simulink model "FMS"  (R2018b)
settings: configuration reference "fms_config" (kept outside this file)
values from neighbouring files (symbols this model uses):
  FMS_EXPORT = Simulink.Parameter(FMS_EXPORT_VALUE)    [fms_model_init.m]
  FMS_PARAM = Simulink.Parameter(FMS_PARAM_VALUE)    [fms_model_init.m]
undefined symbols (not defined in the file or in its folder): actuator_cmd, cmd_mask, ControlMode, ctrl_mode, DiscIntNeverNeededParam, FMS_Cmd, FMS_CONST, home, mode, PilotMode, r_cmd, reset, state, status, timestamp, u_cmd, VehicleState, VehicleStatus, wp_consume, wp_current
libraries: simulink x45, FMT_Model_Lib x35, hdlsllib x2
(part 3 of 3)

== system FMS/FMS Commander/Commander/Arm/Assist/Position/Position Command/Controller/Hold Control/Lateral_Acceleration/L1_Lateral_Acceleration/Included Angle ==
  vec1 : Inport
  vec2 : Inport  Port=2
  2D Cross Product : FMT_Model_Lib/Math/2D Cross Product
      settings: SourceProductName=FMT Toolbox
  Acos : Trigonometry  Operator=acos
  Constant4 : Constant  OutDataTypeStr=single
  Demux : Demux  Outputs=2
  Demux1 : Demux  Outputs=2
  Dot Product : DotProduct  InputSameDT=on  OutDataTypeStr=Inherit: Inherit via internal rule
  Multiply : Product
  Mux : Mux  Inputs=2
  Mux1 : Mux  Inputs=2
  Sign1 : Signum
  Switch2 : Switch  Criteria=u2 ~= 0
  Vector Normalize : FMT_Model_Lib/Math/Vector Normalize
      settings: SourceProductName=FMT Toolbox
  Vector Normalize1 : FMT_Model_Lib/Math/Vector Normalize
      settings: SourceProductName=FMT Toolbox
  angle_rad : Outport
  wires:
  Switch2/1 -> Multiply/2
  Acos/1 -> Multiply/1
  Mux/1 -> Vector Normalize1/1
  vec2/1 -> Demux/1
  Constant4/1 -> Switch2/3
  Demux/1 -> Mux/2
  vec1/1 -> Demux1/1
  Multiply/1 -> angle_rad/1
  2D Cross Product/1 -> Sign1/1
  Vector Normalize/1 -> 2D Cross Product/2, Dot Product/1
  Demux/2 -> Mux/1
  Vector Normalize1/1 -> 2D Cross Product/1, Dot Product/2
  Sign1/1 -> Switch2/2, Switch2/1
  Demux1/2 -> Mux1/1
  Mux1/1 -> Vector Normalize/1
  Demux1/1 -> Mux1/2
  Dot Product/1 -> Acos/1

== matlab function FMS/FMS Commander/Commander/Arm/SubMode/Return/Velocity Commander/L1 Reference WP/NearbyRefWP ==
  data: P output; P2 input; d output; P3 input; L1 input
% Find the reference waypoint when vehicle (P3) is close to target (P2)
%
% If the vehicle is close to target (distance(P2,P3) < L1), select P2 as
% reference waypoint and return the distance, otherwise return -1.
function [P,d] = NearbyRefWP(P2, P3, L1)

P3P2 = P2 - P3;
dis = sqrt(sum(P3P2.^2));

if dis <= L1
    d = dis;
    % select P2 as reference WP
    P = P2;
else
    d = single(-1);
    % unset WP
    P = single([0; 0]);
end

== matlab function FMS/FMS Commander/Commander/Arm/SubMode/Return/Velocity Commander/L1 Reference WP/OutRegionRegWP ==
  data: P1 input; P output; P2 input; P3 input
% Find the reference waypoint when vehicle is out of L1 region near P1P2.
%
% There are three region defined:
%   Region 1: The project point of P3 is lied on left side of P1P2
%   Region 2: The project point of P3 is lied on right side of P1P2
%   Region 3: The project point of P3 is lied on the segment line 
%
%   For the case of region 3, we select the project point as the reference
%   wayspoint. For the case of region 1, we choose P1 as reference waypoint
%   and similarly for the case of region 2, we choose P3 as reference
%   waypoint.
function P = OutRegionRefWP(P1, P2, P3)
% segment line P1P2
P1P2 = P2 - P1;
% segment line P1P3
P1P3 = P3 - P1;

% Define C as the P3 project point on line P1P2.
% Hence, P1C = dot(P1P3, P1P2)/|P1P2| * (P1P2/|P1P2|) = u * P1P2
% where u = dot(P1P3, P1P2) / |P1P2|^2.
u = dot(P1P3, P1P2) / sum(P1P2.^2);

if u <= 0
    % region 1
    P = P1;
elseif u >= 1
    % region 2
    P = P2;
else
    % region 3. C = P1C + P1
    P = u * P1P2 + P1;
end

== stateflow chart FMS/SafeMode ==
  state Other
  state Offboard
  state Mission
  state Position
  state Stabilize
  state Manual
  (junction 21) -> Other
  Other -> (junction 68) : {target_mode = mode;}
  (junction 75) -> (junction 21) [order 2]
  (junction 68) -> (junction 84)
  Offboard -> (junction 78)
  (junction 78) -> (junction 84) [order 1] : [bitget(flag, 4)&&bitget(flag, 5)]
      | {target_mode = PilotMode.Offboard;}
  (junction 75) -> Offboard [order 1] : [mode == PilotMode.Offboard]
  (junction 78) -> (junction 88) [order 2]
  (junction 84) -> (junction 48)
  (junction 1) -> (junction 75) [order 2]
  (junction 1) -> Mission [order 1] : [mode == PilotMode.Mission]
  Mission -> (junction 16)
  (junction 16) -> (junction 48) [order 1] : [bitget(flag, 4)&&bitget(flag, 6)]
      | {target_mode = PilotMode.Mission;}
  (junction 16) -> (junction 88) [order 2]
  (junction 47) -> (junction 1) [order 2]
  (junction 48) -> (junction 51)
  (junction 47) -> Position [order 1] : [mode == PilotMode.Position]
  Position -> (junction 49)
  (junction 49) -> (junction 51) [order 1] : [bitget(flag, 4)&&bitget(flag, 7)]
      | {target_mode = PilotMode.Position;}
  (junction 49) -> (junction 88) [order 2]
  (junction 24) -> (junction 47) [order 2]
  (junction 51) -> (junction 39)
  (junction 88) -> Stabilize
  (junction 24) -> Stabilize [order 1] : [mode == PilotMode.Stabilize]
  Stabilize -> (junction 44)
  (junction 44) -> (junction 39) [order 1] : [bitget(flag, 4)]{target_mode = PilotMode.Stabilize;}
  (junction 44) -> Manual [order 2]
  (junction 10) -> (junction 24) [order 1]
  (junction 39) -> (junction 15)
  (default) -> (junction 10)
  (junction 10) -> Manual [order 2] : [mode == PilotMode.Manual]
  Manual -> (junction 15) : {target_mode = PilotMode.Manual;}
  (junction 41) -> (junction 10)
  (junction 15) -> (junction 40)
  (junction 40) -> (junction 41)
  data: target_mode output; mode input Enum: PilotMode; flag input uint32

== matlab function FMS/FMS Commander/Commander/Arm/SubMode/Return/Velocity Commander/L1 Reference WP/SearchL1RefWP ==
  data: P1 input; P output; P2 input; P3 input; L1 input; u output
% Find reference waypoint (L1RefWP) on the line segment P1P2 which has 
% L1 distance from vehicle position (P3).
%
% The idea is to calculate the intersection point of a circle with L1 radius
% with the line segment P1P2.
%
% Define P = P1 + u * (P2 - P1), where P is the intersection point.
% Goal is calculating the u, where the valid u is between [0, 1].
%
% Input:
%   P1: start point of segment line
%   P2: start point of segment line
%   P3: circle center point, also is known as the vehicle position
%   L1: the L1 distance
% Output:
%   P: L1 reference waypoint
%   u: scale factor (valid between 0 and 1), -1 means no intersection.
function [P, u] = SearchL1RefWP(P1, P2, P3, L1)

% P1 = (x1, y1), P2 = (x2, y2), P3 = (x3, y3)
x1 = P1(1);
y1 = P1(2);
x2 = P2(1);
y2 = P2(2);
x3 = P3(1);
y3 = P3(2);

% The P is on circle and line segment, which yields:
A = (x2 - x1)^2 + (y2 - y1)^2;
B = 2 * ((x2 - x1)*(x1 - x3) + (y2 - y1)*(y1 - y3));
C = x3^2 + y3^2 + x1^2 + y1^2 - 2*(x3*x1 + y3*y1) - L1^2;
% Check root existence confition if B^2 - 4*A*C >= 0
D = B^2 - 4*A*C;
u = single(-1);
P = single([0 0]);

if D > 0
    % D>0 means we have 2 difference roots, % root is valid only if u is in range of [0, 1]
    u1 = (-B + sqrt(D)) / (2*A);
    u2 = (-B - sqrt(D)) / (2*A);
    
    if (u1>=0 && u1<=1) && (u2>=0 && u2<=1)
        % have 2 valid roots, select the one which is closer to P2 (target point)
        if u1 > u2
            u = u1; 
        else
            u = u2;
        end
    elseif (u1>=0 && u1<=1)
        % only 1 root valid, select it
        u = u1;
    elseif (u2>=0 && u2<=1)
        % only 1 root valid, select it
        u = u2;
    else
        % no valid root, which means no intersection point founded.
        return;
    end
elseif D == 0
    % D=0 means only 1 single root
    u1 = -B / (2*A);
    if (u1>=0 && u1<=1)
        % valid root, select it
        u = u1;
    else
        % no valid root, which means no intersection point founded.
        return;
    end
else
    % no valid root, which means no intersection point founded.
    return;
end

% calculate the L1 reference waypoint (P) coordinate
P(1) = x1 + u*(x2 - x1);
P(2) = y1 + u*(y2 - y1);

== matlab function FMS/FMS Commander/Commander/Arm/Auto/Mission/Mission_SubSystem/Velocity Commander/L1 Reference WP/NearbyRefWP ==
  data: P output; P2 input; d output; P3 input; L1 input
% Find the reference waypoint when vehicle (P3) is close to target (P2)
%
% If the vehicle is close to target (distance(P2,P3) < L1), select P2 as
% reference waypoint and return the distance, otherwise return -1.
function [P,d] = NearbyRefWP(P2, P3, L1)

P3P2 = P2 - P3;
dis = sqrt(sum(P3P2.^2));

if dis <= L1
    d = dis;
    % select P2 as reference WP
    P = P2;
else
    d = single(-1);
    % unset WP
    P = single([0; 0]);
end

== matlab function FMS/FMS Commander/Commander/Arm/Auto/Mission/Mission_SubSystem/Velocity Commander/L1 Reference WP/OutRegionRegWP ==
  data: P1 input; P output; P2 input; P3 input
% Find the reference waypoint when vehicle is out of L1 region near P1P2.
%
% There are three region defined:
%   Region 1: The project point of P3 is lied on left side of P1P2
%   Region 2: The project point of P3 is lied on right side of P1P2
%   Region 3: The project point of P3 is lied on the segment line 
%
%   For the case of region 3, we select the project point as the reference
%   wayspoint. For the case of region 1, we choose P1 as reference waypoint
%   and similarly for the case of region 2, we choose P3 as reference
%   waypoint.
function P = OutRegionRefWP(P1, P2, P3)
% segment line P1P2
P1P2 = P2 - P1;
% segment line P1P3
P1P3 = P3 - P1;

% Define C as the P3 project point on line P1P2.
% Hence, P1C = dot(P1P3, P1P2)/|P1P2| * (P1P2/|P1P2|) = u * P1P2
% where u = dot(P1P3, P1P2) / |P1P2|^2.
u = dot(P1P3, P1P2) / sum(P1P2.^2);

if u <= 0
    % region 1
    P = P1;
elseif u >= 1
    % region 2
    P = P2;
else
    % region 3. C = P1C + P1
    P = u * P1P2 + P1;
end

== matlab function FMS/FMS Commander/Commander/Arm/Auto/Mission/Mission_SubSystem/Velocity Commander/L1 Reference WP/SearchL1RefWP ==
  data: P1 input; P output; P2 input; P3 input; L1 input; u output
% Find reference waypoint (L1RefWP) on the line segment P1P2 which has 
% L1 distance from vehicle position (P3).
%
% The idea is to calculate the intersection point of a circle with L1 radius
% with the line segment P1P2.
%
% Define P = P1 + u * (P2 - P1), where P is the intersection point.
% Goal is calculating the u, where the valid u is between [0, 1].
%
% Input:
%   P1: start point of segment line
%   P2: start point of segment line
%   P3: circle center point, also is known as the vehicle position
%   L1: the L1 distance
% Output:
%   P: L1 reference waypoint
%   u: scale factor (valid between 0 and 1), -1 means no intersection.
function [P, u] = SearchL1RefWP(P1, P2, P3, L1)

% P1 = (x1, y1), P2 = (x2, y2), P3 = (x3, y3)
x1 = P1(1);
y1 = P1(2);
x2 = P2(1);
y2 = P2(2);
x3 = P3(1);
y3 = P3(2);

% The P is on circle and line segment, which yields:
A = (x2 - x1)^2 + (y2 - y1)^2;
B = 2 * ((x2 - x1)*(x1 - x3) + (y2 - y1)*(y1 - y3));
C = x3^2 + y3^2 + x1^2 + y1^2 - 2*(x3*x1 + y3*y1) - L1^2;
% Check root existence confition if B^2 - 4*A*C >= 0
D = B^2 - 4*A*C;
u = single(-1);
P = single([0 0]);

if D > 0
    % D>0 means we have 2 difference roots, % root is valid only if u is in range of [0, 1]
    u1 = (-B + sqrt(D)) / (2*A);
    u2 = (-B - sqrt(D)) / (2*A);
    
    if (u1>=0 && u1<=1) && (u2>=0 && u2<=1)
        % have 2 valid roots, select the one which is closer to P2 (target point)
        if u1 > u2
            u = u1; 
        else
            u = u2;
        end
    elseif (u1>=0 && u1<=1)
        % only 1 root valid, select it
        u = u1;
    elseif (u2>=0 && u2<=1)
        % only 1 root valid, select it
        u = u2;
    else
        % no valid root, which means no intersection point founded.
        return;
    end
elseif D == 0
    % D=0 means only 1 single root
    u1 = -B / (2*A);
    if (u1>=0 && u1<=1)
        % valid root, select it
        u = u1;
    else
        % no valid root, which means no intersection point founded.
        return;
    end
else
    % no valid root, which means no intersection point founded.
    return;
end

% calculate the L1 reference waypoint (P) coordinate
P(1) = x1 + u*(x2 - x1);
P(2) = y1 + u*(y2 - y1);

== stateflow chart FMS/FMS Commander/Commander/Arm/Assist/Stabilize/Heading Command/Detect Movement/Motion State ==
  state Hold
    entry:
    state=MotionState.Hold;
  state Move
    entry:
    state=MotionState.Move;
  state Brake
    entry:
    state=MotionState.Brake;
  (default) -> Move
  Hold -> Move : [motion_req==1 ]
  Move -> Brake : [motion_req==0]
  Brake -> Move [order 1] : [motion_req==1]
  Brake -> Hold [order 2] : after(1.5, sec)
  data: state output Enum: MotionState; motion_req input

== stateflow chart FMS/FMS State Machine ==
  state Command_Listener [parallel]
    settings: executionOrder=1
    state Send
      entry:
      % Send command
      M.data=save_cmd;
      send(M);
    state Listen
    state Check
      entry:
      valid_cmd = CheckCmdValid(save_cmd, mode, INS_Out.flag);
    (default) -> Listen
    Send -> Listen
    Listen -> Check : [hasChanged(cmd) && ...
        | cmd ~= FMS_Cmd.None]{save_cmd = cmd;}
    Check -> Listen [order 2]
    Check -> Send [order 1] : [valid_cmd == true]
  state Vehicle [parallel]
    du:
    % if mission data updated, reset waypoint index
    if hasChanged(mission_timestamp)
    wp_consume = 0;
    wp_index = 1;
    end
    settings: executionOrder=4
    state moved = StickMoved(stick_val,pilot_cmd) [function]
    state Arm
      en:
      status = VehicleStatus.Arm;
      state SubMode
        en:
        stick_val = [Pilot_Cmd.stick_yaw; Pilot_Cmd.stick_throttle; Pilot_Cmd.stick_roll; Pilot_Cmd.stick_pitch];
        state Hold
          en:
          state = VehicleState.Hold;
        state Return
          en:
          state = VehicleState.Return;
        SubMode -> Hold [order 1] : M[M.data==FMS_Cmd.Pause]
      state Auto
        state Offboard
          state Loiter
            en:
            state = VehicleState.Hold;
          state Run
            en:
            state = VehicleState.Offboard;
          (default) -> (junction 950)
          (junction 950) -> Vehicle.Arm.Auto.Offboard.Loiter [order 2]
          (junction 950) -> Run [order 1] : [auto_cmd_valid == 1]
          Run -> Vehicle.Arm.Auto.Offboard.Loiter : [auto_cmd_valid == 0]
          Vehicle.Arm.Auto.Offboard.Loiter -> Run : [auto_cmd_valid == 1]
        state Mission
          en:
          % Reference location of latitude and longitude, specified as an m-by-2 array, in degrees
          llo = [INS_Out.lat_0, INS_Out.lon_0] * (180/pi);
          Cmd_In.cur_waypoint =[INS_Out.x_R; INS_Out.y_R; INS_Out.h_R];
          state pos = LLA2FLAT(lla,llo,href,psio) [function]
          state Loiter
            en:
            state = VehicleState.Hold;
          state NextWP
            en:
            if wp_index <= Mission_Data.valid_items
            nav_cmd = Mission_Data.command(wp_index);
            else
            nav_cmd = uint16(NAV_Cmd.None);
            % updated consumed waypoints
            wp_consume = wp_index - 1;
            end
          state Waypoint
            en:
            % Geodetic coordinates (latitude, longitude, and altitude), specified as an m-by-3 array in [degrees degrees meters]
            % Altitude add home(3) here because the altitude when takeoff could be non-zero
            lla = [double(Mission_Data.x(wp_index))*1e-7, double(Mission_Data.y(wp_index))*1e-7, double(-(Mission_Data.z(wp_index) + home(3)))];
            % target waypoint
            Cmd_In.sp_waypoint = LLA2FLAT(lla, llo, 0, 0);
            state = VehicleState.Mission;
          state Return
            en:
            Cmd_In.sp_waypoint = [home(1); home(2); INS_Out.h_R];
            state = VehicleState.Return;
          Mission -> NextWP : [hasChanged(mission_timestamp)]
          (junction 908) -> (junction 910) : {wp_index = wp_index + 1;}
          (junction 910) -> NextWP
          (junction 873) -> (junction 908)
          (default) -> NextWP
          (junction 917) -> Vehicle.Arm.Auto.Mission.Loiter
          (junction 879) -> (junction 873)
          NextWP -> (junction 917) [order 3]
          NextWP -> Waypoint [order 1] : [nav_cmd == NAV_Cmd.Waypoint]
          Waypoint -> (junction 879) : [norm([INS_Out.x_R;INS_Out.y_R]-Cmd_In.sp_waypoint(1:2)) <= accept_radius]
              | {Cmd_In.cur_waypoint = Cmd_In.sp_waypoint;}
          (junction 915) -> (junction 879)
          NextWP -> Vehicle.Arm.Auto.Mission.Return [order 2] : [nav_cmd == NAV_Cmd.Return]
          Vehicle.Arm.Auto.Mission.Return -> (junction 915) : [norm([INS_Out.x_R; INS_Out.y_R]-Cmd_In.sp_waypoint(1:2)) < 0.5]
        state InvalidAutoMode
        (default) -> (junction 43)
        (junction 43) -> Offboard [order 1] : [mode == PilotMode.Offboard]
        (junction 43) -> (junction 134) [order 2]
        (junction 134) -> Mission [order 1] : [mode == PilotMode.Mission]
        (junction 134) -> InvalidAutoMode [order 2]
        InvalidAutoMode -> (junction 370)
      state Assist
        state InvalidAssistMode
        state Stabilize
          en:
          state = VehicleState.Stabilize;
        state Position
          en:
          state = VehicleState.Position;
        (default) -> (junction 190)
        (junction 190) -> (junction 196) [order 2]
        (junction 196) -> InvalidAssistMode [order 2]
        (junction 190) -> Stabilize [order 1] : [mode == PilotMode.Stabilize]
        (junction 196) -> Position [order 1] : [mode == PilotMode.Position]
      state Manual
        state InValidManualMode
        state Manual
          en:
          state = VehicleState.Manual;
        (default) -> (junction 410)
        (junction 410) -> InValidManualMode [order 2]
        (junction 410) -> Vehicle.Arm.Manual.Manual [order 1] : [mode == PilotMode.Manual]
      state InvalidArmMode
      Vehicle.Arm -> Vehicle.Arm.SubMode.Return [order 2] : M[M.data==FMS_Cmd.Return]
          | {Cmd_In.sp_waypoint = [home(1); home(2); single(0)]}
      Hold -> Vehicle.Arm : M[M.data==FMS_Cmd.Continue ...
          | && mode ~= PilotMode.None]
      Auto -> Hold : M[M.data==FMS_Cmd.Pause]
      SubMode -> (junction 117) [order 1] : [StickMoved(stick_val, Pilot_Cmd) && ...
          | mode ~= PilotMode.None]
      Vehicle.Arm -> (junction 117) [order 1] : [hasChanged(mode) && ...
          | mode ~= PilotMode.None]
      (junction 117) -> Auto [order 1] : [getArmMode(mode) == 3]
      (default) -> (junction 117)
      (junction 117) -> (junction 140) [order 2]
      (junction 140) -> Assist [order 1] : [getArmMode(mode)  == 2]
      (junction 140) -> (junction 240) [order 2]
      (junction 240) -> Vehicle.Arm.Manual [order 1] : [getArmMode(mode)  == 1]
      (junction 240) -> InvalidArmMode [order 2]
    state Standby
      en:
      % check if mission takeoff is valid
      if mode==PilotMode.Mission
      if wp_index <= Mission_Data.valid_items > 0
      % set mission takeoff flag, so enter mission mode after 2s
      prep_mission = 1;
      else
      send(DisarmEvent);
      end
      end
      % set current position as home
      home = [INS_Out.x_R; INS_Out.y_R; INS_Out.h_R; INS_Out.psi];
      % enter standby state
      state = VehicleState.Standby;
      status = VehicleStatus.Standby;
      ex:
      % on exit, unset flag
      prep_mission = 0;
    state Disarm
      en:
      state = VehicleState.Disarm;
      status = VehicleStatus.Disarm;
    InValidManualMode -> Vehicle
    Vehicle.Arm.SubMode.Return -> (junction 330) : [norm([INS_Out.x_R,INS_Out.y_R]-[home(1),home(2)]) ...
        | <= accept_radius]
    (junction 330) -> Vehicle.Disarm
    (junction 969) -> Hold
    (junction 968) -> (junction 969) : [pilot_cmd_lost]
    InvalidAssistMode -> Vehicle
    (junction 370) -> Vehicle
    (default) -> Vehicle.Disarm
    Assist -> (junction 968)
    Standby -> Vehicle.Disarm [order 2] : after(10, sec) || DisarmEvent
    Standby -> Vehicle.Arm [order 1] : [ManualArmEvent(Pilot_Cmd) == 1 &&...
        | mode ~= PilotMode.None]
    Vehicle.Disarm -> Standby : M[M.data==FMS_Cmd.PreArm]
    Standby -> Vehicle.Arm [order 4] : [mode == PilotMode.Offboard && ...
        | auto_cmd_valid]
    Vehicle -> Vehicle.Disarm : M[M.data==FMS_Cmd.Disarm]
    Standby -> (junction 903) [order 3] : [duration(prep_mission == 1) >= 2]
    (junction 903) -> Vehicle.Arm
    InvalidArmMode -> Vehicle
  state Combo_Stick [parallel]
    settings: executionOrder=2
    state res = BottomRight(pilot_cmd) [function]
      (default) -> (junction 285) : {res = (pilot_cmd.stick_throttle < -0.8) && ...
          | (pilot_cmd.stick_yaw > 0.8);}
    state Idle
      du:
      bl = BottomLeft(Pilot_Cmd);
      br = BottomRight(Pilot_Cmd);
    state Arm
      en:
      M.data=FMS_Cmd.PreArm;
      send(M);
    state res = BottomLeft(pilot_cmd) [function]
      (default) -> (junction 298) : {res = (pilot_cmd.stick_throttle < -0.8) && ...
          | (pilot_cmd.stick_yaw < -0.8);}
    state Disarm
      en:
      send(DisarmEvent, Vehicle)
    (default) -> Idle
    Combo_Stick.Arm -> Idle : [~BottomRight(Pilot_Cmd)]
    Idle -> Combo_Stick.Arm [order 1] : [duration(br)>1.5]
    Idle -> Combo_Stick.Disarm [order 2] : [duration(bl)>1.5]
    Combo_Stick.Disarm -> Idle : [~BottomLeft(Pilot_Cmd)]
  state Lost_Return [parallel]
    settings: executionOrder=3
    state Lost
      en:
      % check if INS valid to return
      if bitand(INS_Out.flag, 221)
      M.data=FMS_Cmd.Return;
      send(M);
      end
    state Connect
    (default) -> Connect
    Connect -> Lost : [lost_connect]
    Lost -> Connect : [~lost_connect]
  data: cmd_in function_input; mode_in function_input; valid function_output; ins_flag function_input; pilotMode function_input; armMode function_output; pilot_cmd function_input; trigger function_output; stick_val function_input double size=4; moved function_output; pilot_cmd function_input Bus: Pilot_Cmd_Bus size=1; lla function_input double size=[1 3]; llo function_input double size=[1 2]; href function_input double size=1; pos function_output; psio function_input double size=1; res function_output; pilot_cmd function_input; res function_output; pilot_cmd function_input; state output Enum: VehicleState; cmd input; valid_cmd local; M local Enum: FMS_Cmd; mode input; Pilot_Cmd input Bus: Pilot_Cmd_Bus; lost_connect input; pilot_cmd_lost input; INS_Out input Bus: INS_Out_Bus; Mission_Data input Bus: Mission_Data_Bus; home data_store_memory; stick_val local; bl local =false; br local =false; nav_cmd local uint16; wp_consume output uint8 =uint8(0); wp_index output uint8 =uint8(1); Cmd_In output Bus: Commander_In_Bus; mission_timestamp input uint32 =uint32(0); status local Enum: VehicleStatus =VehicleStatus.None; llo local; lla local; save_cmd local Enum: FMS_Cmd; accept_radius input; prep_mission local =0; auto_cmd_valid input
  events: DisarmEvent local FUNCTION_CALL_EVENT
  function valid = CheckCmdValid(cmd_in, mode_in, ins_flag):
    | function valid = CheckCmdValid(cmd_in, mode_in, ins_flag)
    | 
    | % bit1 |    bit2    |    bit3  |   bit4  | bit5  | bit6  |bit7|bit8|bit9
    | % init | standstill | attitude | heading | speed | LLA   | xy | h | h_AGL
    | 
    | valid = false;
    | 
    | if ~bitget(ins_flag, 1)
    |    return; 
    | end
    | 
    | % TODO: Add more checks
    | switch cmd_in
    |     case {FMS_Cmd.Return, FMS_Cmd.Pause}
    |         % these modes need position valid
    |         if bitget(ins_flag, 4) && bitget(ins_flag, 5) && bitget(ins_flag, 7)
    |             valid = true;
    |         end
    |     case FMS_Cmd.PreArm
    |         switch mode_in
    |             case {PilotMode.Position, PilotMode.Offboard}
    |                 if bitget(ins_flag, 4) && bitget(ins_flag, 5) && bitget(ins_flag, 7)
    |                     valid = true;
    |                 end
    |             case PilotMode.Mission
    |                 if bitget(ins_flag, 4) && bitget(ins_flag, 5) && bitget(ins_flag, 6) && bitget(ins_flag, 7)
    |                     valid = true;
    |                 end
    |             case {PilotMode.Stabilize, PilotMode.Manual}
    |                 valid = true;
    |             otherwise
    |                 % do nothing
    |         end
    |     case FMS_Cmd.Continue
    |         if mode_in == PilotMode.Offboard || mode_in == PilotMode.Mission
    |            valid = true; 
    |         end
    |     case FMS_Cmd.Disarm
    |         valid = true;   % always allowed disarm
    |     otherwise
    |         % do nothing
    | end
    | 
    | return;
  function armMode = getArmMode(pilotMode):
    | function armMode = getArmMode(pilotMode)
    | 
    | % Map pilot mode to arm mode
    | switch pilotMode
    |     case PilotMode.Manual
    |         armMode = 1;    % manual
    |     case {PilotMode.Acro, PilotMode.Stabilize, PilotMode.Altitude, PilotMode.Position}
    |         armMode = 2;    % asist
    |     case {PilotMode.Mission, PilotMode.Offboard}
    |         armMode = 3;    % auto
    |     otherwise
    |         armMode = 0;    % unknown
    | end
    | 
    | end
  function trigger = ManualArmEvent(pilot_cmd):
    | function trigger = ManualArmEvent(pilot_cmd)
    | 
    | trigger = 0;
    | 
    | % Map pilot mode to arm mode
    | switch pilot_cmd.mode
    |     case {PilotMode.Manual, PilotMode.Stabilize, PilotMode.Position}
    |         if pilot_cmd.stick_throttle > 0
    |             trigger = 1;
    |         end
    |     otherwise
    |         % do nothing
    | end
    | 
    | end

== matlab function FMS/FMS Commander/Commander/Arm/Auto/Offboard/Rotation_Command/Velocity Commander/L1 Reference WP/NearbyRefWP ==
  data: P output; P2 input; d output; P3 input; L1 input
% Find the reference waypoint when vehicle (P3) is close to target (P2)
%
% If the vehicle is close to target (distance(P2,P3) < L1), select P2 as
% reference waypoint and return the distance, otherwise return -1.
function [P,d] = NearbyRefWP(P2, P3, L1)

P3P2 = P2 - P3;
dis = sqrt(sum(P3P2.^2));

if dis <= L1
    d = dis;
    % select P2 as reference WP
    P = P2;
else
    d = single(-1);
    % unset WP
    P = single([0; 0]);
end

== matlab function FMS/FMS Commander/Commander/Arm/Auto/Offboard/Rotation_Command/Velocity Commander/L1 Reference WP/OutRegionRegWP ==
  data: P1 input; P output; P2 input; P3 input
% Find the reference waypoint when vehicle is out of L1 region near P1P2.
%
% There are three region defined:
%   Region 1: The project point of P3 is lied on left side of P1P2
%   Region 2: The project point of P3 is lied on right side of P1P2
%   Region 3: The project point of P3 is lied on the segment line 
%
%   For the case of region 3, we select the project point as the reference
%   wayspoint. For the case of region 1, we choose P1 as reference waypoint
%   and similarly for the case of region 2, we choose P3 as reference
%   waypoint.
function P = OutRegionRefWP(P1, P2, P3)
% segment line P1P2
P1P2 = P2 - P1;
% segment line P1P3
P1P3 = P3 - P1;

% Define C as the P3 project point on line P1P2.
% Hence, P1C = dot(P1P3, P1P2)/|P1P2| * (P1P2/|P1P2|) = u * P1P2
% where u = dot(P1P3, P1P2) / |P1P2|^2.
u = dot(P1P3, P1P2) / sum(P1P2.^2);

if u <= 0
    % region 1
    P = P1;
elseif u >= 1
    % region 2
    P = P2;
else
    % region 3. C = P1C + P1
    P = u * P1P2 + P1;
end

== matlab function FMS/FMS Commander/Commander/Arm/Auto/Offboard/Rotation_Command/Velocity Commander/L1 Reference WP/SearchL1RefWP ==
  data: P1 input; P output; P2 input; P3 input; L1 input; u output
% Find reference waypoint (L1RefWP) on the line segment P1P2 which has 
% L1 distance from vehicle position (P3).
%
% The idea is to calculate the intersection point of a circle with L1 radius
% with the line segment P1P2.
%
% Define P = P1 + u * (P2 - P1), where P is the intersection point.
% Goal is calculating the u, where the valid u is between [0, 1].
%
% Input:
%   P1: start point of segment line
%   P2: start point of segment line
%   P3: circle center point, also is known as the vehicle position
%   L1: the L1 distance
% Output:
%   P: L1 reference waypoint
%   u: scale factor (valid between 0 and 1), -1 means no intersection.
function [P, u] = SearchL1RefWP(P1, P2, P3, L1)

% P1 = (x1, y1), P2 = (x2, y2), P3 = (x3, y3)
x1 = P1(1);
y1 = P1(2);
x2 = P2(1);
y2 = P2(2);
x3 = P3(1);
y3 = P3(2);

% The P is on circle and line segment, which yields:
A = (x2 - x1)^2 + (y2 - y1)^2;
B = 2 * ((x2 - x1)*(x1 - x3) + (y2 - y1)*(y1 - y3));
C = x3^2 + y3^2 + x1^2 + y1^2 - 2*(x3*x1 + y3*y1) - L1^2;
% Check root existence confition if B^2 - 4*A*C >= 0
D = B^2 - 4*A*C;
u = single(-1);
P = single([0 0]);

if D > 0
    % D>0 means we have 2 difference roots, % root is valid only if u is in range of [0, 1]
    u1 = (-B + sqrt(D)) / (2*A);
    u2 = (-B - sqrt(D)) / (2*A);
    
    if (u1>=0 && u1<=1) && (u2>=0 && u2<=1)
        % have 2 valid roots, select the one which is closer to P2 (target point)
        if u1 > u2
            u = u1; 
        else
            u = u2;
        end
    elseif (u1>=0 && u1<=1)
        % only 1 root valid, select it
        u = u1;
    elseif (u2>=0 && u2<=1)
        % only 1 root valid, select it
        u = u2;
    else
        % no valid root, which means no intersection point founded.
        return;
    end
elseif D == 0
    % D=0 means only 1 single root
    u1 = -B / (2*A);
    if (u1>=0 && u1<=1)
        % valid root, select it
        u = u1;
    else
        % no valid root, which means no intersection point founded.
        return;
    end
else
    % no valid root, which means no intersection point founded.
    return;
end

% calculate the L1 reference waypoint (P) coordinate
P(1) = x1 + u*(x2 - x1);
P(2) = y1 + u*(y2 - y1);

== stateflow chart FMS/FMS Commander/Commander/Arm/Assist/Position/Position Command/Detect Movement/Motion State ==
  state Hold
    entry:
    state=MotionState.Hold;
  state Move
    entry:
    state=MotionState.Move;
  state Brake
    entry:
    state=MotionState.Brake;
  (default) -> Move
  Hold -> Move : [motion_req==1 ]
  Move -> Brake : [motion_req==0]
  Brake -> Move [order 1] : [motion_req==1]
  Brake -> Hold [order 2] : after(1.5, sec)
  data: state output Enum: MotionState; motion_req input

== matlab function FMS/FMS Commander/Commander/Arm/Assist/Position/Position Command/Controller/Hold Control/L1_Reference_WP/SearchL1RefWP ==
  data: c input; P output; p0 input; n input; L1 input; t output
function [P, t] = SearchL1RefWP(c, p0, n, L1)

m = p0 - c;
A = 1;  % dot(n,n) = 1
B = 2*dot(n, m);
C = dot(m, m) - L1^2;

% Check root existence confition if B^2 - 4*A*C >= 0
D = B^2 - 4*A*C;

t = single(-1);
P = single([0;0]);

if D > 0
    % D>0 means we have 2 difference roots, % root is valid only if u is in range of [0, 1]
    u1 = (-B + sqrt(D)) / (2*A);
    u2 = (-B - sqrt(D)) / (2*A);
    
    % have 2 valid roots, select the one which is farthur
    if u1 > u2
        t = u1; 
    else
        t = u2;
    end
    
    % calculate the L1 reference waypoint (P) coordinate
    P = p0 + t*n;
elseif D == 0
    t = -B / (2*A);
    
    % calculate the L1 reference waypoint (P) coordinate
    P = p0 + t*n;
else
    % only 1 root or no valid root, use other logic to find WP.
    return;
end

== matlab function FMS/FMS Commander/Commander/Arm/Assist/Position/Position Command/Controller/Hold Control/L1_Reference_WP/OutRegionRefWP ==
  data: c input; P output; p0 input; n input
function P  = OutRegionRefWP(c, p0, n)

P1P3 = c - p0;

% Define C as the P3 (vehicle) project point on ray.
% Hence, P1C = dot(P1P3, P1P2)/|P1P2| * (P1P2/|P1P2|) = t * P1P2
% where t = dot(P1P3, P1P2) / |P1P2|^2. Choose P1P2 as a normalized vector,
% therefore |P1P2| = 1, yield t = dot(P1P3, n)
t = dot(P1P3, n);
C = p0 + t*n;

% Now we calculate the distance forward from C with 30deg
d1 = norm(C - c);
d2 = d1 * tan(pi/6);

% Calculate the final waypoint
P = p0 + (t+d2)*n;
